simulink model "lab2_v10_all"  (R2026b)
settings: Solver=ode45  StopTime=12  MaxStep=0.005
settings Model: Creator=polina  LastModifiedBy=polina

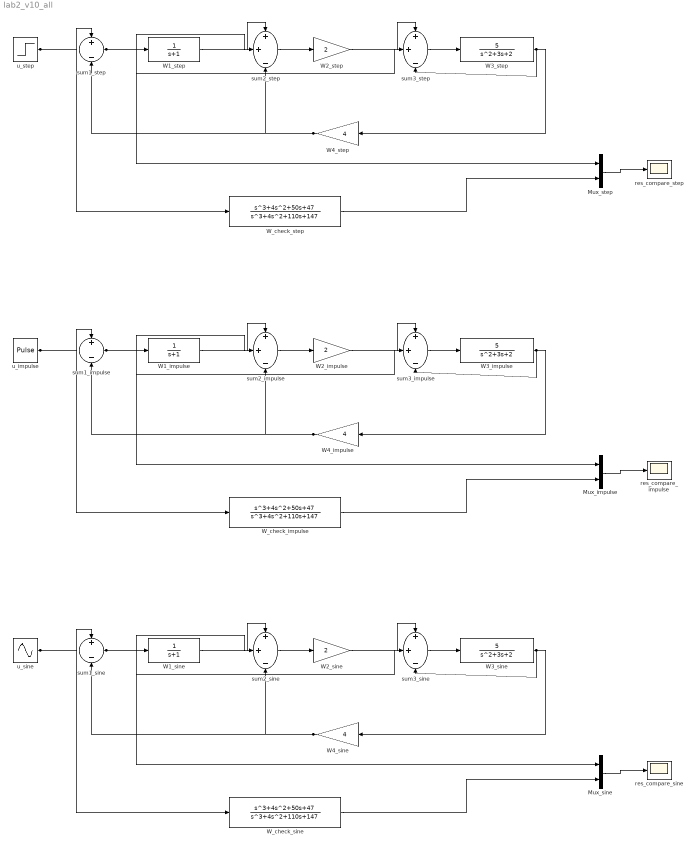
== system lab2_v10_all ==
  Mux_impulse : Mux  Inputs=2
  Mux_sine : Mux  Inputs=2
  Mux_step : Mux  Inputs=2
  W1_impulse : TransferFcn  Denominator=[1 1]
  W1_sine : TransferFcn  Denominator=[1 1]
  W1_step : TransferFcn  Denominator=[1 1]
  W2_impulse : Gain  Gain=2
  W2_sine : Gain  Gain=2
  W2_step : Gain  Gain=2
  W3_impulse : TransferFcn  Numerator=[5]  Denominator=[1 3 2]
  W3_sine : TransferFcn  Numerator=[5]  Denominator=[1 3 2]
  W3_step : TransferFcn  Numerator=[5]  Denominator=[1 3 2]
  W4_impulse : Gain  Gain=4
  W4_sine : Gain  Gain=4
  W4_step : Gain  Gain=4
  W_check_impulse : TransferFcn  Numerator=[1 4 50 47]  Denominator=[1 4 110 147]
  W_check_sine : TransferFcn  Numerator=[1 4 50 47]  Denominator=[1 4 110 147]
  W_check_step : TransferFcn  Numerator=[1 4 50 47]  Denominator=[1 4 110 147]
  res_compare_impulse : Scope
  res_compare_sine : Scope
  res_compare_step : Scope
  sum1_impulse : Sum  Inputs=+-
  sum1_sine : Sum  Inputs=+-
  sum1_step : Sum  Inputs=+-
  sum2_impulse : Sum  Inputs=++-
  sum2_sine : Sum  Inputs=++-
  sum2_step : Sum  Inputs=++-
  sum3_impulse : Sum  Inputs=++-
  sum3_sine : Sum  Inputs=++-
  sum3_step : Sum  Inputs=++-
  u_impulse : DiscretePulseGenerator  PulseType=Time based  Amplitude=20  Period=20  PulseWidth=0.25  PhaseDelay=1
  u_sine : Sin  Frequency=2  SampleTime=0
  u_step : Step  SampleTime=0
  wires:
  u_step/1 -> sum1_step/1, W_check_step/1
  sum1_step/1 -> W1_step/1, sum2_step/2, sum3_step/2, Mux_step/1
  W1_step/1 -> sum2_step/1
  sum2_step/1 -> W2_step/1
  W2_step/1 -> sum3_step/1
  sum3_step/1 -> W3_step/1
  W3_step/1 -> sum3_step/3, W4_step/1
  W4_step/1 -> sum1_step/2, sum2_step/3
  W_check_step/1 -> Mux_step/2
  Mux_step/1 -> res_compare_step/1
  u_impulse/1 -> sum1_impulse/1, W_check_impulse/1
  sum1_impulse/1 -> W1_impulse/1, sum2_impulse/2, sum3_impulse/2, Mux_impulse/1
  W1_impulse/1 -> sum2_impulse/1
  sum2_impulse/1 -> W2_impulse/1
  W2_impulse/1 -> sum3_impulse/1
  sum3_impulse/1 -> W3_impulse/1
  W3_impulse/1 -> sum3_impulse/3, W4_impulse/1
  W4_impulse/1 -> sum1_impulse/2, sum2_impulse/3
  W_check_impulse/1 -> Mux_impulse/2
  Mux_impulse/1 -> res_compare_impulse/1
  u_sine/1 -> sum1_sine/1, W_check_sine/1
  sum1_sine/1 -> W1_sine/1, sum2_sine/2, sum3_sine/2, Mux_sine/1
  W1_sine/1 -> sum2_sine/1
  sum2_sine/1 -> W2_sine/1
  W2_sine/1 -> sum3_sine/1
  sum3_sine/1 -> W3_sine/1
  W3_sine/1 -> sum3_sine/3, W4_sine/1
  W4_sine/1 -> sum1_sine/2, sum2_sine/3
  W_check_sine/1 -> Mux_sine/2
  Mux_sine/1 -> res_compare_sine/1
